simulink model "UAV_Sim_Ninad"  (R2026b)
settings: Solver=VariableStepAuto  StopTime=10
undefined symbols (not defined in the file or in its folder): quad_m, W
libraries: aerolibanimutils x1, uavutilslib x1
settings Model: Creator=Ninad  LastModifiedBy=Ninad

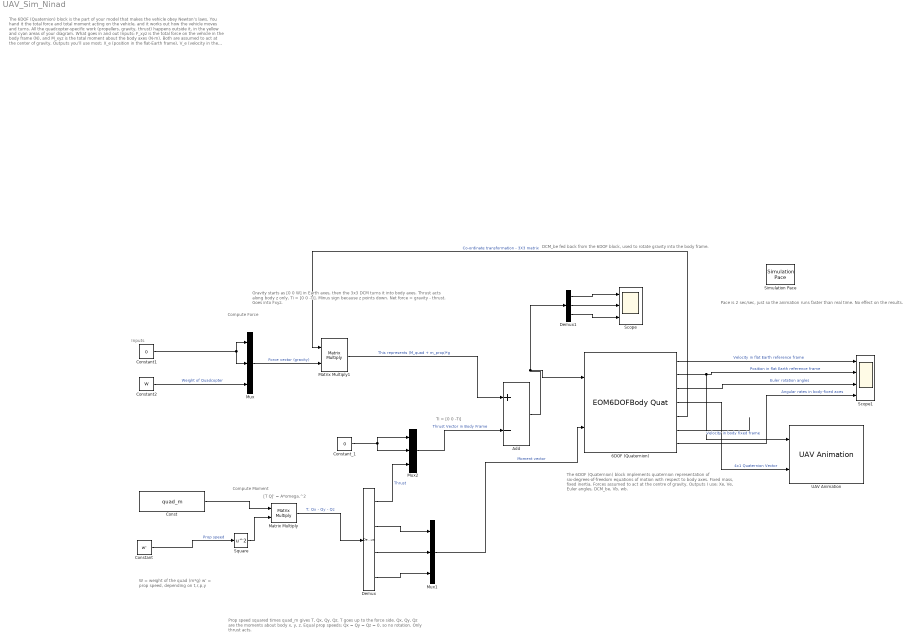
== system UAV_Sim_Ninad ==
  note: Pace is 2 sec/sec, just so the animation runs faster than real time. No effect on the results.
  note: DCM_be fed back from the 6DOF block, used to rotate gravity into the body frame.
  note: Prop speed squared times quad_m gives T, Qx, Qy, Qz. T goes up to the force side. Qx, Qy, Qz are the moments about body x, y, z. Equal prop speeds: Qx = Qy = Qz = 0, so no rotation. Only thrust acts.
  note: Gravity starts as [0 0 W] in Earth axes, then the 3x3 DCM turns it into body axes. Thrust acts along body z only, Ti = [0 0 -Ti]. Minus sign because z points down. Net force = gravity - thrust. Goes into Fxyz.
  note: W = weight of the quad (m*g)
      | w' = prop speed, depending on t,r,p,y
  note: Compute Moment
  note: Inputs
  note: [T Q]' = A*omega.^2
  note: The 6DOF (Quaternion) block implements quaternion representation of six-degrees-of-freedom equations of motion with respect to body axes.
      |
      | Fixed mass, fixed inertia. Forces assumed to act at the centre of gravity. Outputs I use: Xe, Ve, Euler angles, DCM_be, Vb, wb.
  note: Ti = [0 0 -Ti]
  note: Compute Force
  note: The 6DOF (Quaternion) block is the part of your model that makes the vehicle obey Newton’s laws. You hand it the total force and total moment acting on the vehicle, and it works out how the vehicle moves and turns. All the quadcopter-specific work (propellers, gravity, thrust) happens outside it, in the yellow and cyan areas of your diagram.
      | What goes in and out
      | Inputs: F_xyz is the total force on the vehicle in the body frame (N), and M_xyz is the total moment about the body axes (N·m). Both are assumed to act at the center of gravity.
      | Outputs you’ll use most: X_e (position in the flat-Earth frame), V_e (velocity in the Earth frame), φθψ (Euler angles), q (the quaternion), DCM_be (the matrix that converts Earth-frame vectors to body-frame), V_b (body-frame velocity) and ω_b (body angular rates).
      | Inside the block dialog: mass, inertia matrix, units, and initial position, velocity, attitude and rates. These are what make it your quad rather than a generic body.
      | What it integrates internally
      | Translation: dV_b/dt = F/m − ω × V_b . The cross-product term appears because the body frame itself is rotating.
      | Rotation: dω/dt = I⁻¹ (M − ω × Iω) .
      | Attitude: the quaternion rate matrix in your screenshot, with a small correction term that keeps the quaternion’s norm at 1.
      | Position: rotate the body velocity back into the Earth frame and integrate.
      | Use the quaternion or DCM_be for anything downstream. The Euler angles are for plotting only, since they become singular at ±90° pitch.
      | Frame convention. The flat-Earth frame is NED, so z points down. Altitude is −z , and your height plot will look inverted unless you negate it. That also explains the “NED” confusion in the YouTube comments.
      | Reading your replica diagram :
      | Compute Force: gravity starts as a vector in the Earth frame, [0; 0; W] with W = m·g . The matrix multiply by DCM_be converts it to the body frame, which is why the DCM output loops back to the top of the diagram. Thrust is built as a vector along the body z-axis. Because z points down, thrust “up” is negative, which is why it enters the sum with a minus sign. The sum gives F_xyz .
      | Compute Moment: propeller speed is squared, and quad_m (a constants matrix from the propeller model) converts ω² into thrust T and torque Q . Those feed the moment vector. This diagram uses one lumped propeller speed, so it can hover and yaw but can’t pitch or roll yet. Differential thrust across four rotors comes in module 5.
      | Right side: the scopes just display outputs, and the 3D drone block is visualization only. Add it last.
      | Build order, with a done-when for each step
      | Place the 6DOF (Quaternion) block from Aerospace Blockset → Equations of Motion → 6DOF and set its mass, inertia and initial conditions. Done when it runs with zero force and moment and nothing moves.
      | Add gravity (Earth-frame vector, multiplied by DCM_be ) as the only force. Done when the quad free-falls and the z output matches ½gt² .
      | Add the thrust vector [0; 0; −T] . Done when setting T = W makes it hover with a constant z.
      | Add the propeller-speed path ( ω² into quad_m , giving T and Q). Done when a hover prop speed, ω = sqrt(W / k_T) , holds the quad steady.
      | Add the moment path and the scopes. Done when changing Q makes the yaw angle change and nothing else.
  6DOF (Quaternion) : EOM6DOFBodyQuat
  Add : Sum  Inputs=+-
  Const : Constant  Value=quad_m
  Constant : Constant  Value=w'
  Constant1 : Constant  Value=0
  Constant2 : Constant  Value=W
  Constant_1 : Constant  Value=0  OutDataTypeStr=Inherit: Inherit via back propagation
  Demux : Demux
  Demux1 : Demux  Outputs=3
  Matrix Multiply : Product  Multiplication=Matrix(*)
  Matrix Multiply1 : Product  Multiplication=Matrix(*)
  Mux : Mux  Inputs=3
  Mux1 : Mux  Inputs=3
  Mux2 : Mux  Inputs=3
  Scope : Scope  NumInputPorts=3
  Scope1 : Scope  NumInputPorts=4
  Simulation Pace : aerolibanimutils/Simulation Pace  SimulationPace=2  SleepMode=Auto  OutputPaceError=off  SampleTime=1/30
  Square : Math  Operator=square
  UAV Animation : uavutilslib/UAV Animation  NumUAV=1  DynamicUAVConfig=off  UAVType=Multirotor  UAVSize=1  UAVColor=[1 0 0]  UAVTrajectoryAlpha=1  AlwaysShowAnimation=on  AxisLimits=[-Inf Inf;-Inf Inf;-Inf Inf]  TrajectoryBufferSize=100000  InertialZDirection=Down  RotationFormat=Quaternion  DrawMarkers=off  SampleTime=-1
  wires:
  Const/1 -> Matrix Multiply/1
  Constant/1 -> Square/1  "Prop speed"
  Square/1 -> Matrix Multiply/2
  Mux/1 -> Matrix Multiply1/2  "Force vector (gravity)"
  Constant1/1 -> Mux/2, Mux/1
  Constant2/1 -> Mux/3  "Weight of Quadcopter"
  Matrix Multiply1/1 -> Add/1  "This represents (M_quad + m_prop)*g"
  Matrix Multiply/1 -> Demux/1  "T; Qx - Qy - Qz"
  Demux/2 -> Mux1/1
  Demux/3 -> Mux1/2
  Demux/4 -> Mux1/3
  Mux1/1 -> 6DOF (Quaternion)/2  "Moment vector"
  Constant_1/1 -> Mux2/2, Mux2/1
  Demux/1 -> Mux2/3  "Thrust"
  Mux2/1 -> Add/2  "Thrust Vector in Body Frame"
  Add/1 -> Demux1/1, 6DOF (Quaternion)/1
  6DOF (Quaternion)/1 -> Scope1/1  "Velocity in flat Earth reference frame"
  6DOF (Quaternion)/2 -> UAV Animation/1, Scope1/2  "Position in flat Earth reference frame"
  6DOF (Quaternion)/3 -> Scope1/3  "Euler rotation angles"
  6DOF (Quaternion)/7 -> Scope1/4  "Angular rates in body-fixed axes"
  6DOF (Quaternion)/4 -> UAV Animation/2  "4x1 Quaternion Vector"
  6DOF (Quaternion)/6 -> ?  "Velocity in body fixed frame"
  6DOF (Quaternion)/5 -> Matrix Multiply1/1  "Co-ordinate transformation - 3X3 matrix"
  Demux1/1 -> Scope/1
  Demux1/2 -> Scope/2
  Demux1/3 -> Scope/3
